simulink model "stereo_camera_q_dot"  (R2025b)
settings: Solver=FixedStepDiscrete  StartTime=0  StopTime=inf  FixedStep=Ts  RelTol=1e-3
InitFcn:
  | % 获取当前.slx模型所在文件夹
  | model_path = fileparts(which(gcs));
  | % 向上跳转、拼接目标函数所在文件夹（根据你的目录调整）
  | func_folder = fullfile(model_path,'..', 'config');
  | % 添加到搜索路径
  | addpath(func_folder);
  | % 执行初始化函数
  | init_stereo_camera_q_dot_tracking;
undefined symbols (not defined in the file or in its folder): camera_velocity_feedback_timeout_sec, controller_enable, cx, cy, data, data_SL_Info, depth_deadband, depth_gain, depth_rate_max, ekf_gate_threshold, enable_ekf_feedforward, enable_proportional, fx, fy, joint_acceleration_limit, joint_nominal_configuration, joint_position_max, joint_position_min, joint_soft_margin, joint_state_timeout_sec, joint_velocity_limit, k_ff, Kpx, Kpy, measurement_reset_timeout, P0, Publish, Q_ekf, R_ekf, required_valid_frames, ros, ros2lib, singularity_sigma_stop, singularity_sigma_warn, Subscribe, target_timeout_sec, task_velocity_filter_tau, Ts, visual_damping_max, visual_damping_min, visual_min_depth, Z_hat, z_ref
libraries: robotmaniplib x2
(part 2 of 2)

== matlab function stereo_camera_q_dot/Planar Target KF and Task Command/KF and Task Command Core ==
  data: T_camera2base input; z_meas input size=[2 1]; ekf_state output size=[4 1]; e input size=[2 1]; safe_valid input size=1; target_is_new input; R_ekf input size=[2 2]; P0 input size=[4 4]; Q_ekf input size=[4 4]; parameters input size=[11 1]; ekf_covariance output size=[4 4]; v_target_hat output size=[2 1]; v_p output size=[2 1]; v_ff output size=[2 1]; v_task_raw output; v_issued output size=[2 1]; camera_velocity output size=[6 1]; control_active output; acceleration_active output; ekf_initialized output size=1; innovation_nis output size=1; measurement_accepted output size=1; controller_ok output size=1; required_valid_frames input; measurement_reset_timeout input; target_visible input; z input
function [ekf_state,ekf_covariance,v_target_hat,v_p,v_ff,v_task_raw,v_issued,camera_velocity,control_active,acceleration_active,ekf_initialized,innovation_nis,measurement_accepted,controller_ok] = fcn( ...
T_camera2base,z_meas,e,safe_valid,target_is_new,R_ekf,P0,Q_ekf,parameters,required_valid_frames,measurement_reset_timeout,target_visible,z)
%#codegen
% 四状态匀速 KF：[X_B;Y_B;Vx_B;Vy_B]。
% 原消息、目标、P/FF 和总控制使能关系保持不变。
% v_task_raw 是未滤波、未限幅的二维相机平移速度请求。
% v_issued 是经过任务空间低通后的二维速度指令。

persistent x_hat P e_hold z_hold time_since_accepted initialized
persistent valid_streak ekf_ready time_since_visible target_tracking_active
persistent v_issued_hold

if isempty(initialized)
x_hat=zeros(4,1); P=P0; e_hold=zeros(2,1); z_hold=0.0;
time_since_accepted=0.0; initialized=false;
valid_streak=0.0; ekf_ready=false;
time_since_visible=inf; target_tracking_active=false;
v_issued_hold=zeros(2,1);
end

ekf_state=x_hat; ekf_covariance=P; v_target_hat=zeros(2,1);
v_p=zeros(2,1); v_ff=zeros(2,1); v_task_raw=zeros(2,1);
v_issued=zeros(2,1); camera_velocity=zeros(6,1);
control_active=false; acceleration_active=false;
ekf_initialized=initialized && ekf_ready; innovation_nis=NaN;
measurement_accepted=false; controller_ok=false;

if numel(parameters)<11
x_hat=zeros(4,1); P=P0; e_hold=zeros(2,1); z_hold=0.0;
time_since_accepted=0.0; initialized=false; valid_streak=0.0;
ekf_ready=false; time_since_visible=inf; target_tracking_active=false;
v_issued_hold=zeros(2,1);
ekf_state=x_hat; ekf_covariance=P; ekf_initialized=false; return;
end

Ts=parameters(1); Z_hat=parameters(2); Kpx=parameters(3); Kpy=parameters(4);
k_ff=parameters(5); gate=parameters(6);
enable_p=parameters(7)>0.5; enable_ff=parameters(8)>0.5;
controller_enable=parameters(9)>0.5;
target_lost_timeout=parameters(10);
task_velocity_filter_tau=parameters(11);

if target_lost_timeout<=0.0, target_lost_timeout=0.10; end

safe_valid=safe_valid>0.5; target_visible=target_visible>0.5;
target_is_new=target_is_new>0.5;
required_valid_frames=max(1.0,floor(required_valid_frames));

parameter_ok=all(isfinite(parameters(1:11))) && ...
isfinite(required_valid_frames) && isfinite(measurement_reset_timeout) && ...
Ts>0.0 && Z_hat>0.0 && gate>0.0 && task_velocity_filter_tau>=0.0 && ...
measurement_reset_timeout>=Ts && target_lost_timeout>=Ts && ...
isequal(size(R_ekf),[2 2]) && isequal(size(P0),[4 4]) && ...
isequal(size(Q_ekf),[4 4]) && all(isfinite(R_ekf(:))) && ...
all(isfinite(P0(:))) && all(isfinite(Q_ekf(:)));

if ~parameter_ok
x_hat=zeros(4,1); P=P0; e_hold=zeros(2,1); z_hold=0.0;
time_since_accepted=0.0; initialized=false; valid_streak=0.0;
ekf_ready=false; time_since_visible=inf; target_tracking_active=false;
v_issued_hold=zeros(2,1);
ekf_state=x_hat; ekf_covariance=P; ekf_initialized=false; return;
end

if ~(isfinite(z_hold) && z_hold>0.0)
z_hold=max(Z_hat,0.10);
end

F=[1 0 Ts 0;0 1 0 Ts;0 0 1 0;0 0 0 1];
H=[1 0 0 0;0 1 0 0]; I4=eye(4);

pose_matrix_ok=isequal(size(T_camera2base),[4 4]) && ...
all(isfinite(T_camera2base(:)));
R_base_camera=eye(3); t_base_camera=zeros(3,1); pose_ok=false;

if pose_matrix_ok
R_candidate=T_camera2base(1:3,1:3);
t_candidate=T_camera2base(1:3,4);
pose_ok=norm(R_candidate'*R_candidate-eye(3),'fro')<1e-3 && ...
abs(det(R_candidate)-1.0)<1e-3 && ...
norm(T_camera2base(4,:)-[0 0 0 1])<1e-6 && ...
all(isfinite(t_candidate));
if pose_ok, R_base_camera=R_candidate; t_base_camera=t_candidate; end
end

measurement_vectors_ok=numel(z_meas)==2 && numel(e)==2 && ...
all(isfinite(z_meas(:))) && all(isfinite(e(:)));
vision_safe=safe_valid && measurement_vectors_ok;

if ~vision_safe
time_since_visible=inf; target_tracking_active=false; e_hold=zeros(2,1);
elseif target_is_new && target_visible
time_since_visible=0.0; target_tracking_active=true; e_hold=reshape(e,2,1);
if isfinite(z) && z>1e-4, z_hold=z; end
else
time_since_visible=min(time_since_visible+Ts,target_lost_timeout+Ts);
if time_since_visible>=target_lost_timeout
target_tracking_active=false; e_hold=zeros(2,1);
end
end

measurement_available=vision_safe && target_is_new && target_visible && ...
pose_ok && isfinite(z) && z>1e-4;
z_base=zeros(2,1); R_measurement_base=R_ekf;

if measurement_available
p_target_camera=[z_meas(1);z_meas(2);z];
p_target_base=R_base_camera*p_target_camera+t_base_camera;
z_base=p_target_base(1:2);
measurement_rotation=R_base_camera(1:2,1:2);
R_measurement_base=measurement_rotation*R_ekf*measurement_rotation';
R_measurement_base=0.5*(R_measurement_base+R_measurement_base');
measurement_available=all(isfinite(z_base(:))) && ...
all(isfinite(R_measurement_base(:)));
end

if ~initialized
if measurement_available
x_hat=[z_base(1);z_base(2);0;0]; P=P0;
initialized=true; measurement_accepted=true;
end
else
x_pred=F*x_hat; P_pred=F*P*F'+Q_ekf; P_pred=0.5*(P_pred+P_pred');
x_hat=x_pred; P=P_pred;

if measurement_available
innovation=z_base-H*x_pred; S=H*P_pred*H'+R_measurement_base;
if all(isfinite(S(:))) && rcond(S)>1e-12
innovation_nis=innovation'*(S\innovation);
else
innovation_nis=inf;
end

if isfinite(innovation_nis) && innovation_nis<=gate
K=(P_pred*H')/S; x_hat=x_pred+K*innovation; A=I4-K*H;
P=A*P_pred*A'+K*R_measurement_base*K';
P=0.5*(P+P'); measurement_accepted=true;
end
end
end

if measurement_accepted
time_since_accepted=0.0;
valid_streak=min(valid_streak+1.0,required_valid_frames);
if valid_streak>=required_valid_frames, ekf_ready=true; end

else
if target_is_new && ~ekf_ready, valid_streak=0.0; end
time_since_accepted=time_since_accepted+Ts;
end

ekf_ok=all(isfinite(x_hat(:))) && all(isfinite(P(:))) && ...
all(diag(P)>=0.0) && norm(P-P','fro')<1e-6;

if time_since_accepted>=measurement_reset_timeout || ~ekf_ok
x_hat=zeros(4,1); P=P0; time_since_accepted=0.0; initialized=false;
valid_streak=0.0; ekf_ready=false; measurement_accepted=false;
end

ekf_state=x_hat; ekf_covariance=P;

if initialized && ekf_ready
v_target_hat=x_hat(3:4);
else
v_target_hat=zeros(2,1); ekf_state(3:4)=zeros(2,1);
end

ekf_initialized=initialized && ekf_ready;

if controller_enable && enable_p && vision_safe && target_tracking_active
v_p=z_hold*[Kpx*e_hold(1);Kpy*e_hold(2)];
else
v_p=zeros(2,1);
end

v_target_camera_xy=zeros(2,1);

if initialized && ekf_ready && pose_ok
v_target_base_3d=[x_hat(3);x_hat(4);0];
v_target_camera_3d=R_base_camera'*v_target_base_3d;
v_target_camera_xy=v_target_camera_3d(1:2);
end

if controller_enable && enable_ff && vision_safe && ...
initialized && ekf_ready && pose_ok
v_ff=k_ff*v_target_camera_xy;
else
v_ff=zeros(2,1);
end

v_task_raw=v_p+v_ff;

control_active=controller_enable && vision_safe && ...
((enable_p && target_tracking_active) || ...
(enable_ff && initialized && ekf_ready && pose_ok));

if control_active
filter_alpha=Ts/(task_velocity_filter_tau+Ts);
v_issued_hold=v_issued_hold+filter_alpha*(v_task_raw-v_issued_hold);
else
v_issued_hold=zeros(2,1);
end

v_issued=v_issued_hold;
camera_velocity=[v_issued;0;0;0;0];
acceleration_active=false;

controller_ok=all(isfinite(v_p(:))) && all(isfinite(v_ff(:))) && ...
all(isfinite(v_task_raw(:))) && all(isfinite(v_issued(:)));

if ~controller_ok
v_p=zeros(2,1); v_ff=zeros(2,1); v_task_raw=zeros(2,1);
v_issued_hold=zeros(2,1); v_issued=zeros(2,1);
camera_velocity=zeros(6,1); control_active=false; e_hold=zeros(2,1);
time_since_visible=inf; target_tracking_active=false;
end
end

== matlab function stereo_camera_q_dot/Redundant Visual Velocity Solver ==
  data: v_issued input; qdot_raw output; e input; z input; J_camera input; q input; safe_valid input; control_active input; controller_ok input; kinematics_valid input; solver_parameters input; q_nominal input; q_min input; q_max input; sigma_min output; damping_used output; singularity_scale output; solver_valid output
function [qdot_raw,sigma_min,damping_used,singularity_scale,solver_valid] = fcn( ...
v_issued,e,z,J_camera,q,safe_valid,control_active,controller_ok, ...
kinematics_valid,solver_parameters,q_nominal,q_min,q_max)
%#codegen
% v_issued：经过任务空间低通后的二维相机平移速度指令。
% J_camera：相机光学坐标系表达、顺序为 [vx;vy;vz;wx;wy;wz]。
%
% 任务优先级（严格降级，后一级不干扰前一级）：
%   P1 图像居中（2 维）：始终执行。
%   P2 深度定点（1 维）：在 P1 的零空间里执行，把深度调到 z_ref。
%   P3 无：本版本不做主动避奇异；q_nominal 端口保留备用。
%
% 本次改动：
%   1) 奇异度判据改用“任务雅可比” [J_image;J_depth]（3x7）的最小奇异值，
%      不再使用 6x7 相机雅可比的第 6 个奇异值；
%   2) 奇异缩放只作用于 P1，不再把深度任务一起清零；
%   3) 删除“回归名义构型 + 软限位回避”的零空间种子（其增益原本为 1e-6，
%      等于未接入），关节限位安全由 Final Joint Command Guard 负责；
%   4) 深度由“安全区推回”改为“定点 z_ref + 死区 + 速率上限”；
%   5) 深度伪逆增加可用性保护，避免分母退化时命令被放大；
%   6) 深度层补偿 P1 图像任务已造成的深度速度，只求解剩余深度残差。
%
% solver_parameters 顺序：
%   1 阻尼下限  2 阻尼上限  3 sigma_stop  4 sigma_warn
%   5 z_ref     6 深度死区  7 depth_gain  8 depth_rate_max  9 minimum_depth
%
% 注意：启用 EKF 前馈后，需要额外给深度补一个“时效”门，否则目标不可见时
% 深度任务可能继续使用历史深度；当前依靠 control_active 的可见性约束。

persistent feature_hold depth_hold
if isempty(depth_hold)
feature_hold=zeros(2,1); depth_hold=0.50;
end

qdot_raw=zeros(7,1); sigma_min=0.0; damping_used=0.0;
singularity_scale=0.0; solver_valid=false;

q=reshape(q,7,1); q_nominal=reshape(q_nominal,7,1);
q_min=reshape(q_min,7,1); q_max=reshape(q_max,7,1);

input_ok=numel(v_issued)==2 && numel(e)==2 && ...
isequal(size(J_camera),[6 7]) && numel(solver_parameters)>=9 && ...
all(isfinite(v_issued(:))) && all(isfinite(e(:))) && ...
all(isfinite(J_camera(:))) && all(isfinite(q(:))) && ...
all(isfinite(q_nominal(:))) && all(isfinite(q_min(:))) && ...
all(isfinite(q_max(:))) && all(q_max>q_min) && ...
all(isfinite(solver_parameters(1:9)));

if ~input_ok
feature_hold=zeros(2,1); depth_hold=0.50; return;
end

lambda_min=solver_parameters(1); lambda_max=solver_parameters(2);
sigma_stop=solver_parameters(3); sigma_warn=solver_parameters(4);
z_ref=solver_parameters(5); depth_deadband=solver_parameters(6);
depth_gain=solver_parameters(7); depth_rate_max=solver_parameters(8);
minimum_depth=solver_parameters(9);

parameter_ok=lambda_min>0.0 && lambda_max>=lambda_min && ...
sigma_stop>=0.0 && sigma_warn>sigma_stop && ...
z_ref>minimum_depth && depth_deadband>=0.0 && ...
depth_gain>=0.0 && depth_rate_max>0.0 && minimum_depth>0.0;

if ~parameter_ok
feature_hold=zeros(2,1); depth_hold=0.50; return;
end

if safe_valid && isfinite(z) && z>minimum_depth
feature_hold=reshape(e,2,1); depth_hold=z;
elseif ~safe_valid
feature_hold=zeros(2,1); depth_hold=max(z_ref,minimum_depth);
end

x=feature_hold(1); y=feature_hold(2); Z=max(depth_hold,minimum_depth);

% ---- 任务雅可比：P1 图像居中 2 行 + P2 深度 1 行 ----
L=[-1.0/Z 0 x/Z x*y -(1.0+x*x) y; ...
0 -1.0/Z y/Z 1.0+y*y -x*y -x];
J_image=L*J_camera;

L_depth=[0 0 -1.0 -Z*y Z*x 0];
J_depth=L_depth*J_camera;

% ---- 奇异度：用任务雅可比（3x7）的最小奇异值 ----
% 这两个量只依赖 J_camera 与 x、y、Z，不依赖阻尼，因此不会和下面形成循环。
% 阈值很小时本段不改变原有行为（singularity_scale 恒为 1）。
singular_values=svd([J_image;J_depth]);
sigma_min=min(singular_values);

if sigma_min<=sigma_stop
singularity_scale=0.0; damping_used=lambda_max;
elseif sigma_min>=sigma_warn
singularity_scale=1.0; damping_used=lambda_min;
else
ratio=(sigma_min-sigma_stop)/(sigma_warn-sigma_stop);
singularity_scale=ratio*ratio*(3.0-2.0*ratio);
damping_used=lambda_max-(lambda_max-lambda_min)*singularity_scale;
end

solver_valid=isfinite(sigma_min) && isfinite(damping_used) && ...
isfinite(singularity_scale);

if ~solver_valid
qdot_raw=zeros(7,1); return;
end

if ~(safe_valid && control_active && controller_ok && kinematics_valid)
qdot_raw=zeros(7,1); return;
end

% ---- P1：图像居中 ----
normal_matrix=J_image*J_image'+damping_used*damping_used*eye(2);

if ~(all(isfinite(normal_matrix(:))) && rcond(normal_matrix)>1e-12)
solver_valid=false; qdot_raw=zeros(7,1); return;
end

J_image_damped=J_image'/normal_matrix;
feature_rate_command=-(reshape(v_issued,2,1)/Z);
qdot_task=J_image_damped*feature_rate_command;
N_image=eye(7)-J_image_damped*J_image;

% ---- P2：深度定点，在 P1 的零空间内 ----
depth_error=z_ref-Z;
depth_rate_command=0.0;

if abs(depth_error)>depth_deadband
depth_rate_command=depth_gain*depth_error;
end

depth_rate_command=min(max(depth_rate_command,-depth_rate_max),depth_rate_max);

% P2 只补偿 P1 执行后剩余的深度速度：
%   深度期望速度 - P1 已造成的深度速度 = P2 需要完成的残差。
% 这样即使深度处于死区，P2 也会抵消图像跟踪引起的已知深度漂移。
qdot_primary=singularity_scale*qdot_task;
depth_rate_from_primary=J_depth*qdot_primary;
depth_rate_residual=depth_rate_command-depth_rate_from_primary;

% 高速跟踪时 P1 可能造成较大的深度速度。P1 优先，P2 的补偿能力
% 仍限制在 depth_rate_max 内，避免为了守住深度而产生过大的关节命令。
depth_rate_residual=min(max(depth_rate_residual,-depth_rate_max),depth_rate_max);

J_depth_null=J_depth*N_image;
depth_denominator=J_depth_null*J_depth_null'+ ...
damping_used*damping_used;

% 可用性保护：剩余自由度里深度方向几乎做不动时不动作。
% 1e-2 是相对 |J_depth| 的保护阈值，不是调参量。
depth_avail_ratio=1e-2;
depth_available=norm(J_depth_null)>depth_avail_ratio*norm(J_depth);

qdot_depth=zeros(7,1);

if abs(depth_rate_residual)>1e-9 && depth_available && ...
isfinite(depth_denominator) && depth_denominator>0.0
qdot_depth=N_image*J_depth'*(depth_rate_residual/depth_denominator);
end

% ---- 合成：P1 优先，P2 在 P1 零空间中完成深度速度残差 ----
qdot_raw=qdot_primary+qdot_depth;

solver_valid=all(isfinite(qdot_raw(:)));
if ~solver_valid, qdot_raw=zeros(7,1); end
end

== matlab function stereo_camera_q_dot/Final Joint Command Guard ==
  data: qdot_raw input; qdot_command output; q input; safe_valid input; control_active input; solver_valid input; guard_parameters input; qdot_limit input; qddot_limit input; q_min input; q_max input; velocity_scale output; acceleration_scale output; position_scale output; guard_valid output
function [qdot_command,velocity_scale,acceleration_scale,position_scale,guard_valid] = fcn( ...
qdot_raw,q,safe_valid,control_active,solver_valid,guard_parameters, ...
qdot_limit,qddot_limit,q_min,q_max)
%#codegen
% 全系统最终关节命令处理：
% 整体速度缩放 -> 逐关节软位置边界 -> 整体加速度缩放。
% 接近上限只限制正速度，接近下限只限制负速度，其他关节正常运动。
% 任务空间低通已在前级控制器中完成，本模块不再重复低通。

persistent previous_command initialized
if isempty(initialized)
previous_command=zeros(7,1); initialized=true;
end

qdot_command=zeros(7,1); velocity_scale=0.0; acceleration_scale=0.0;
position_scale=0.0; guard_valid=false;
qdot_raw=reshape(qdot_raw,7,1); q=reshape(q,7,1);
qdot_limit=reshape(qdot_limit,7,1);
qddot_limit=reshape(qddot_limit,7,1);
q_min=reshape(q_min,7,1); q_max=reshape(q_max,7,1);

input_ok=numel(guard_parameters)==2 && ...
all(isfinite(qdot_raw(:))) && all(isfinite(q(:))) && ...
all(isfinite(qdot_limit(:))) && all(qdot_limit>0.0) && ...
all(isfinite(qddot_limit(:))) && all(qddot_limit>0.0) && ...
all(isfinite(q_min(:))) && all(isfinite(q_max(:))) && ...
all(q_max>q_min) && all(isfinite(guard_parameters(1:2)));
if ~input_ok
previous_command=zeros(7,1); return;
end

Ts=guard_parameters(1); soft_margin=guard_parameters(2);
parameter_ok=Ts>0.0 && soft_margin>0.0;
if ~parameter_ok
previous_command=zeros(7,1); return;
end

target_velocity=zeros(7,1);
% 使能或数据失效时把目标速度置零，并通过加速度限制缓降。
if safe_valid && control_active && solver_valid
target_velocity=qdot_raw;
end

% 整体速度缩放：任一关节达到速度限值时，7维方向同比例保留。
maximum_velocity_ratio=max(abs(target_velocity)./qdot_limit);
velocity_scale=1.0/max(1.0,maximum_velocity_ratio);
velocity_limited=target_velocity*velocity_scale;

% 逐关节限制靠近位置边界时的向外速度，不影响返回速度和其他关节。
position_scale=1.0;
for joint_index=1:7
local_scale=1.0;

if velocity_limited(joint_index)>0.0
distance_to_limit=q_max(joint_index)-q(joint_index);
local_scale=min(max(distance_to_limit/soft_margin,0.0),1.0);
elseif velocity_limited(joint_index)<0.0
distance_to_limit=q(joint_index)-q_min(joint_index);
local_scale=min(max(distance_to_limit/soft_margin,0.0),1.0);
end

velocity_limited(joint_index)=velocity_limited(joint_index)*local_scale;
position_scale=min(position_scale,local_scale);
end

% 整体加速度缩放：限制本周期7维速度变化，保持变化方向。
delta_velocity=velocity_limited-previous_command;
maximum_acceleration_ratio=max(abs(delta_velocity)./(qddot_limit*Ts));
acceleration_scale=1.0/max(1.0,maximum_acceleration_ratio);
qdot_command=previous_command+delta_velocity*acceleration_scale;

% 到达位置边界后，只禁止对应关节继续向外，允许其返回。
for joint_index=1:7
if q(joint_index)>=q_max(joint_index) && qdot_command(joint_index)>0.0
qdot_command(joint_index)=0.0;
position_scale=0.0;
elseif q(joint_index)<=q_min(joint_index) && qdot_command(joint_index)<0.0
qdot_command(joint_index)=0.0;
position_scale=0.0;
end
end

guard_valid=all(isfinite(qdot_command(:)));
if guard_valid
previous_command=qdot_command;
else
qdot_command=zeros(7,1); previous_command=zeros(7,1);
velocity_scale=0.0; acceleration_scale=0.0; position_scale=0.0;
end
end

== matlab function stereo_camera_q_dot/Joint Velocity Publisher/Pack Seven Joint Velocities ==
  data: qdot_command input; data output; current_length output; received_length output
function [data,current_length,received_length] = fcn(qdot_command)
%#codegen
data=zeros(128,1);
data(1:7)=reshape(qdot_command,7,1);
current_length=uint32(7);
received_length=uint32(7);
end

== matlab function stereo_camera_q_dot/Target ROS2 Subscriber/Unpack ==
  data: data input; target_data output size=[4 1]; is_new input size=1; t input size=1; target_count output size=1; target_age output size=1
function [target_data,target_count,target_age] = fcn(data,is_new,t)
%#codegen
% target_data = [valid; u; v; depth_m]

persistent last_data last_count last_time

if isempty(last_count)
    last_data  = zeros(4,1);
    last_count = 0.0;
    last_time  = -1.0e6;
end

if is_new
    n = numel(data);

    last_data = zeros(4,1);

    if n >= 1, last_data(1) = data(1); end  % valid
    if n >= 2, last_data(2) = data(2); end  % u
    if n >= 3, last_data(3) = data(3); end  % v
    if n >= 4, last_data(4) = data(4); end  % depth_m

    last_count = double(n);
    last_time  = t;
end

target_data  = last_data;
target_count = last_count;
target_age   = max(0.0,t-last_time);
end

== matlab function stereo_camera_q_dot/Kinematics Feedback/MATLAB Function ==
  data: J_camera_base_wv input; camera_twist_measured output; qdot_measured input; T_camera2base input; joint_count input; joint_age input; feedback_timeout input; kinematics_valid output; T_camera2base_out output; J_camera output
function [camera_twist_measured,kinematics_valid,T_camera2base_out,J_camera] = fcn( ...
    J_camera_base_wv,qdot_measured,T_camera2base,joint_count,joint_age,feedback_timeout)
%#codegen
% Get Jacobian 输出为 Base 表达的 [omega;v]。
% 本函数输出相机光学坐标系表达的 [v;omega] 和完整 6x7 Jacobian。

camera_twist_measured = zeros(6,1);
kinematics_valid = false;
T_camera2base_out = eye(4);
J_camera = zeros(6,7);
qdot_measured = reshape(qdot_measured,7,1);

input_ok = joint_count >= 7 && isfinite(joint_age) && ...
    isfinite(feedback_timeout) && feedback_timeout > 0.0 && ...
    joint_age >= 0.0 && joint_age <= feedback_timeout && ...
    all(isfinite(qdot_measured(:))) && ...
    isequal(size(J_camera_base_wv),[6 7]) && ...
    all(isfinite(J_camera_base_wv(:))) && ...
    isequal(size(T_camera2base),[4 4]) && ...
    all(isfinite(T_camera2base(:)));

if ~input_ok
    return;
end

R_base_camera = T_camera2base(1:3,1:3);
pose_ok = norm(R_base_camera'*R_base_camera-eye(3),'fro') < 1e-3 && ...
    abs(det(R_base_camera)-1.0) < 1e-3 && ...
    norm(T_camera2base(4,:)-[0 0 0 1]) < 1e-6;
if ~pose_ok
    return;
end

% 先把 [omega;v] 改成统一的 [v;omega]。
J_base_vw = J_camera_base_wv([4 5 6 1 2 3],:);
R_camera_base = R_base_camera';
rotation6 = [R_camera_base zeros(3);zeros(3) R_camera_base];

% Jacobian 已经是在 camera_link 原点计算，因此这里只改变表达坐标系，
% 不再重复加入相机安装平移偏置。
J_camera = rotation6*J_base_vw;
camera_twist_measured = J_camera*qdot_measured;
T_camera2base_out = T_camera2base;

kinematics_valid = all(isfinite(J_camera(:))) && ...
    all(isfinite(camera_twist_measured(:)));
if ~kinematics_valid
    J_camera = zeros(6,7);
    camera_twist_measured = zeros(6,1);
end
end

== matlab function stereo_camera_q_dot/Joint State ROS2 Subscriber/Unpack ==
  data: name input; name_info input; position input; position_info input; joint_position output size=[7 1]; velocity input; velocity_info input; is_new input size=1; t input size=1; joint_count output size=1; joint_velocity output size=[7 1]; joint_age output size=1
function [joint_position,joint_count,joint_velocity,joint_age] = fcn( ...
    name,name_info,position,position_info,velocity,velocity_info,is_new,t)
%#codegen
% ROS JointState 的 name、position、velocity 使用相同索引。
% 仅当 fr3_joint1...fr3_joint7 均唯一存在且数组索引完整时才更新输出。

persistent last_q last_dq last_count last_time
if isempty(last_count)
    last_q=zeros(7,1); last_dq=zeros(7,1);
    last_count=0.0; last_time=-1.0e6;
end

if is_new
    last_q=zeros(7,1); last_dq=zeros(7,1);
    last_count=0.0; last_time=t;

    name_count=min(double(name_info.CurrentLength),double(numel(name)));
    position_count=min(double(position_info.CurrentLength),double(numel(position)));
    velocity_count=min(double(velocity_info.CurrentLength),double(numel(velocity)));

    arrays_not_truncated = ...
        double(name_info.CurrentLength)==double(name_info.ReceivedLength) && ...
        double(position_info.CurrentLength)==double(position_info.ReceivedLength) && ...
        double(velocity_info.CurrentLength)==double(velocity_info.ReceivedLength);
    message_shape_ok = arrays_not_truncated && name_count>=7.0 && ...
        position_count>=7.0 && velocity_count>=7.0;

    if message_shape_ok
        expected_names=uint8([ ...
            'fr3_joint1';'fr3_joint2';'fr3_joint3';'fr3_joint4'; ...
            'fr3_joint5';'fr3_joint6';'fr3_joint7']);
        matched=false(7,1); source_order=zeros(7,1); names_valid=true;

        for source_index=1:numel(name)
            if double(source_index)<=name_count
                character_count=min( ...
                    double(name(source_index).data_SL_Info.CurrentLength), ...
                    double(numel(name(source_index).data)));
                string_not_truncated = ...
                    double(name(source_index).data_SL_Info.CurrentLength)== ...
                    double(name(source_index).data_SL_Info.ReceivedLength);

                if string_not_truncated && character_count==10.0
                    for expected_index=1:7
                        same_name=true;
                        for character_index=1:10
                            if name(source_index).data(character_index)~= ...
                                    expected_names(expected_index,character_index)
                                same_name=false;
                            end
                        end

                        if same_name
                            if matched(expected_index)
                                names_valid=false;
                            else
                                matched(expected_index)=true;
                                source_order(expected_index)=double(source_index);
                            end
                        end
                    end
                end
            end
        end

        names_valid=names_valid && all(matched);
        indices_valid=names_valid && all(source_order>=1.0) && ...
            all(source_order<=position_count) && ...
            all(source_order<=velocity_count);

        if indices_valid
            for joint_index=1:7
                source_index=source_order(joint_index);
                last_q(joint_index)=position(source_index);
                last_dq(joint_index)=velocity(source_index);
            end

            values_valid=all(isfinite(last_q(:))) && all(isfinite(last_dq(:)));
            if values_valid
                last_count=7.0;
            else
                last_q=zeros(7,1); last_dq=zeros(7,1);
            end
        end
    end
end

joint_position=last_q; joint_count=last_count;
joint_velocity=last_dq; joint_age=max(0.0,t-last_time);
end

== matlab function stereo_camera_q_dot/Message Validation/Validate ==
  data: target_data input size=[4 1]; safe_valid output size=1; target_visible output size=1; target_count input size=1; joint_position input size=[7 1]; joint_count input size=1; joint_velocity input size=[7 1]; u output size=1; v output size=1; z output; joint_position_out output size=[7 1]; joint_velocity_out output size=[7 1]; joint_age input size=1; target_age input; joint_state_timeout_sec input; target_timeout_sec input
function [ ...
    safe_valid, ...
    target_visible, ...
    u, ...
    v, ...
    z, ...
    joint_position_out, ...
    joint_velocity_out] = fcn( ...
    target_data, ...
    target_count, ...
    joint_position, ...
    joint_count, ...
    joint_velocity, ...
    joint_age, ...
    target_age, ...
    joint_state_timeout_sec, ...
    target_timeout_sec)
%#codegen
%
% target_data：
%   (1) valid
%   (2) u，pixel
%   (3) v，pixel
%   (4) z，m

%% 1. 初始化输出

safe_valid = false;
target_visible = false;

u = 0.0;
v = 0.0;
z = 0.0;

joint_position_out = zeros(7,1);
joint_velocity_out = zeros(7,1);

%% 2. 视觉消息有效性

target_count_valid = ...
    isfinite(target_count) && ...
    target_count >= 4;

target_data_finite = ...
    all(isfinite(target_data(1:4)));

target_age_valid = ...
    isfinite(target_age) && ...
    isfinite(target_timeout_sec) && ...
    target_timeout_sec > 0.0 && ...
    target_age >= 0.0 && ...
    target_age <= target_timeout_sec;

vision_data_ok = ...
    target_count_valid && ...
    target_data_finite && ...
    target_age_valid;

%% 3. 当前是否检测到目标

target_visible = ...
    vision_data_ok && ...
    target_data(1) > 0.5;

%% 4. 关节状态有效性

joint_count_valid = ...
    isfinite(joint_count) && ...
    joint_count >= 7;

joint_pos_finite = ...
    numel(joint_position) >= 7 && ...
    all(isfinite(joint_position(1:7)));

joint_vel_finite = ...
    numel(joint_velocity) >= 7 && ...
    all(isfinite(joint_velocity(1:7)));

joint_age_valid = ...
    isfinite(joint_age) && ...
    isfinite(joint_state_timeout_sec) && ...
    joint_state_timeout_sec > 0.0 && ...
    joint_age >= 0.0 && ...
    joint_age <= joint_state_timeout_sec;

joint_ok = ...
    joint_count_valid && ...
    joint_pos_finite && ...
    joint_vel_finite && ...
    joint_age_valid;

%% 5. 输出目标数据

if target_visible
    u = target_data(2);
    v = target_data(3);
    z = target_data(4);
end

%% 6. 输出关节数据

if joint_ok
    joint_position_out = ...
        reshape(joint_position(1:7),7,1);

    joint_velocity_out = ...
        reshape(joint_velocity(1:7),7,1);
end

%% 7. 整体安全使能

safe_valid = ...
    vision_data_ok && ...
    joint_ok;

end
